simulink model "Simulink"  (R2023a)
settings: Solver=VariableStepAuto  StartTime=0.0  StopTime=1  RelTol=1e-3
libraries: dspmlti4 x10
settings Model: Creator=Hasan  LastModifiedBy=Hasan
settings DataIOCC: ReturnWorkspaceOutputs=off
settings DebuggingCC: ParameterPrecisionLossMsg=none

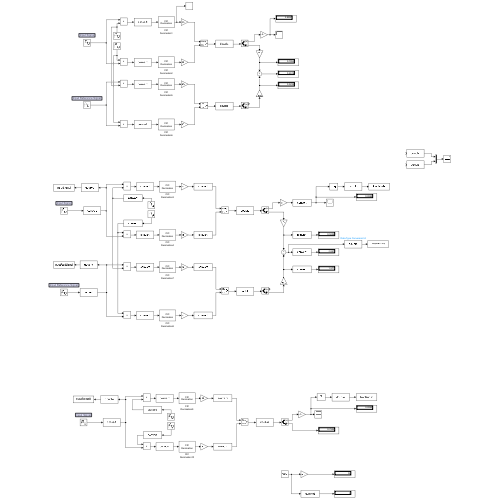
[thumbnail: Simulink's stored preview of the top-level diagram]
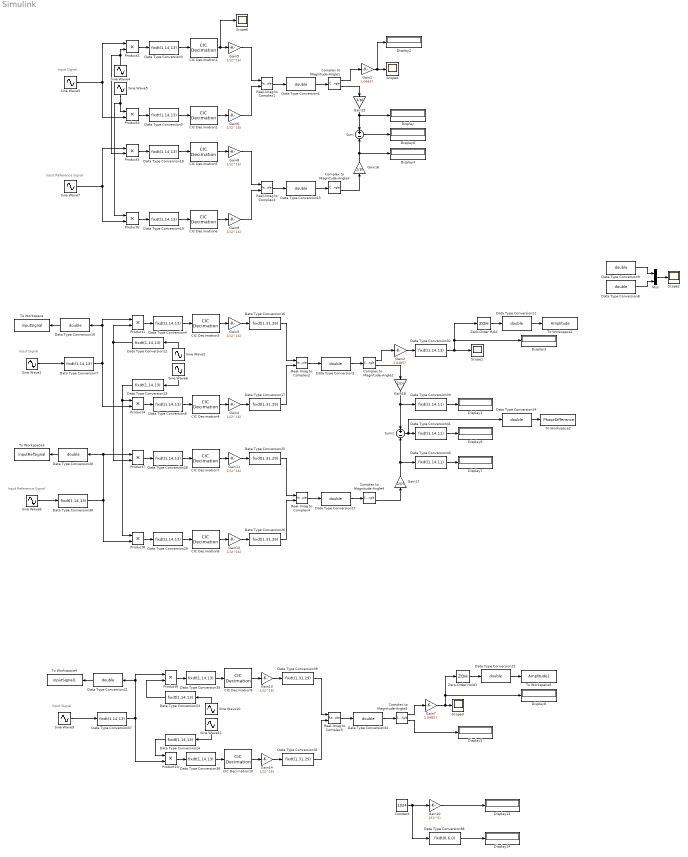
== system Simulink ==
  note: Input Signal
  note: Input Signal
  note: Input Reference Signal
  note: Input Reference Signal
  note: Input Signal
  CIC Decimation{1..2,4..6,8,10} (7 alike) : dspmlti4/CIC Decimation  filtFrom=Dialog parameters  filtobj=CICDECIM  ftype=Decimator  R=50  M=1  N=3  filterInternals=Full precision  BPS=[16 16 16 16]  FLPS=0  outputWordLength=50  outputFracLength=0  launchFVT=off  framing=Maintain input frame rate  RateOptions=Allow multirate processing
      settings: LibrarySourceBlock=|
      | dsphdlsupportfiltering/CIC
      | Decimation
  CIC Decimation3 : dspmlti4/CIC Decimation  filtFrom=Dialog parameters  filtobj=CICDECIM  ftype=Decimator  R=50  M=1  N=3  filterInternals=Full precision  BPS=[16 16 16 16]  FLPS=0  outputWordLength=14  outputFracLength=0  launchFVT=off  framing=Maintain input frame rate  RateOptions=Allow multirate processing
      settings: LibrarySourceBlock=|
      | dsphdlsupportfiltering/CIC
      | Decimation
  CIC Decimation7 : dspmlti4/CIC Decimation  filtFrom=Dialog parameters  filtobj=CICDECIM  ftype=Decimator  R=50  M=1  N=3  filterInternals=Full precision  BPS=[16 16 16 16]  FLPS=0  outputWordLength=14  outputFracLength=0  launchFVT=off  framing=Maintain input frame rate  RateOptions=Allow multirate processing
      settings: LibrarySourceBlock=|
      | dsphdlsupportfiltering/CIC
      | Decimation
  CIC Decimation9 : dspmlti4/CIC Decimation  filtFrom=Dialog parameters  filtobj=CICDECIM  ftype=Decimator  R=50  M=1  N=3  filterInternals=Full precision  BPS=[16 16 16 16]  FLPS=0  outputWordLength=14  outputFracLength=0  launchFVT=off  framing=Maintain input frame rate  RateOptions=Allow multirate processing
      settings: LibrarySourceBlock=|
      | dsphdlsupportfiltering/CIC
      | Decimation
  Complex to Magnitude-Angle{1..5} (5 alike) : ComplexToMagnitudeAngle
  Constant : Constant  Value=1024
  Data Type Conversion{1..2,8..11,14..15,20..22,27,34} (13 alike) : DataTypeConversion  OutDataTypeStr=double  SaturateOnIntegerOverflow=off  RndMeth=Floor
  Data Type Conversion{3..7,12..13,18..19,23..24,28..30,32,35..37} (18 alike) : DataTypeConversion  OutDataTypeStr=fixdt(1,14,13)  SaturateOnIntegerOverflow=off  RndMeth=Floor
  Data Type Conversion{16..17,25..26,31,39} (6 alike) : DataTypeConversion  OutDataTypeStr=fixdt(1,31,29)  SaturateOnIntegerOverflow=off  RndMeth=Floor
  Data Type Conversion33 : DataTypeConversion  OutDataTypeStr=fixdt(1,14,11)  SaturateOnIntegerOverflow=off  RndMeth=Floor
  Data Type Conversion38 : DataTypeConversion  OutDataTypeStr=fixdt(0,6,0)  SaturateOnIntegerOverflow=off  RndMeth=Floor
  Data Type Conversion40 : DataTypeConversion  OutDataTypeStr=fixdt(1,14,11)  SaturateOnIntegerOverflow=off  RndMeth=Floor
  Data Type Conversion41 : DataTypeConversion  OutDataTypeStr=fixdt(1,14,11)  SaturateOnIntegerOverflow=off  RndMeth=Floor
  Display{,1..9,13..14} (12 alike) : Display
  Gain1 : Gain  Gain=1.04857
  Gain10 : Gain  Gain=1/(2^5)  ParamDataTypeStr=double  OutDataTypeStr=double
  Gain{3..6,8..9,11..14} (10 alike) : Gain  Gain=1/(2^16)
  Gain15 : Gain  Gain=1/pi
  Gain16 : Gain  Gain=1/pi
  Gain17 : Gain  Gain=1/pi  ParamDataTypeStr=fixdt(1,14,12)  OutDataTypeStr=fixdt(1,29,25)
  Gain18 : Gain  Gain=1/pi  ParamDataTypeStr=fixdt(1,14,12)  OutDataTypeStr=fixdt(1,29,25)
  Gain2 : Gain  Gain=1.04857  ParamDataTypeStr=fixdt(1,14,12)  OutDataTypeStr=fixdt(1,29,25)
  Gain7 : Gain  Gain=1.04857  ParamDataTypeStr=fixdt(1,14,12)  OutDataTypeStr=fixdt(1,45,41)
  Mux : Mux  Inputs=2
  Product{1..10} (10 alike) : Product
  Real-Imag to Complex{1..5} (5 alike) : RealImagToComplex
  Scope{1..4,6} (5 alike) : Scope
  Sine Wave1 : Sin  Amplitude=.9  Frequency=2*pi*60e6  Phase=pi/6  SampleTime=1/150e6
  Sine Wave10 : Sin  Amplitude=0.9999  Frequency=2*pi*60e6  SampleTime=1/150e6
  Sine Wave11 : Sin  Amplitude=0.9999  Frequency=2*pi*60e6  Phase=pi/2  SampleTime=1/150e6
  Sine Wave2 : Sin  Amplitude=0.9999  Frequency=2*pi*60e6  SampleTime=1/150e6
  Sine Wave3 : Sin  Amplitude=0.9  Frequency=2*pi*60e6  Phase=pi/4  SampleTime=1/150e6
  Sine Wave4 : Sin  Amplitude=.9999  Frequency=2*pi*60e6  SampleTime=1/150e6
  Sine Wave5 : Sin  Amplitude=0.99999  Frequency=2*pi*60e6  Phase=pi/2  SampleTime=1/150e6
  Sine Wave6 : Sin  Amplitude=0.9999  Frequency=2*pi*60e6  Phase=pi/2  SampleTime=1/150e6
  Sine Wave7 : Sin  Amplitude=0.9  Frequency=2*pi*60e6  Phase=pi/6  SampleTime=1/150e6
  Sine Wave8 : Sin  Amplitude=0.9  Frequency=2*pi*60e6  Phase=pi/2  SampleTime=1/150e6
  Sine Wave9 : Sin  Amplitude=0.9  Frequency=2*pi*60e6  Phase=pi/4  SampleTime=1/150e6
  Sum : Sum  Inputs=+|-
  Sum1 : Sum  Inputs=+|-
  To Workspace : ToWorkspace  VariableName=inputSignal  SaveFormat=Timeseries  SampleTime=-1
  To Workspace1 : ToWorkspace  VariableName=Amplitude  SaveFormat=Timeseries  SampleTime=-1
  To Workspace2 : ToWorkspace  VariableName=PhaseDifference  SaveFormat=Timeseries  SampleTime=-1
  To Workspace3 : ToWorkspace  VariableName=inputRefSignal  SaveFormat=Timeseries  SampleTime=-1
  To Workspace4 : ToWorkspace  VariableName=inputSignal1  SaveFormat=Timeseries  SampleTime=-1
  To Workspace5 : ToWorkspace  VariableName=Amplitude1  SaveFormat=Timeseries  SampleTime=-1
  Zero-Order Hold : ZeroOrderHold  SampleTime=1/150e6
  Zero-Order Hold1 : ZeroOrderHold  SampleTime=1/150e6
  wires:
  Real-Imag to Complex1/1 -> Data Type Conversion1/1
  CIC Decimation1/1 -> Scope6/1, Gain5/1
  Sine Wave3/1 -> Product2/1, Product3/2
  Sine Wave4/1 -> Product5/2, Product2/2
  Product3/1 -> Data Type Conversion5/1
  Data Type Conversion3/1 -> CIC Decimation1/1
  Data Type Conversion5/1 -> CIC Decimation2/1
  CIC Decimation2/1 -> Gain6/1
  Data Type Conversion1/1 -> Complex to Magnitude-Angle1/1
  Complex to Magnitude-Angle1/1 -> Gain1/1
  Complex to Magnitude-Angle2/1 -> Gain2/1
  Data Type Conversion2/1 -> Complex to Magnitude-Angle2/1
  Data Type Conversion6/1 -> CIC Decimation4/1
  Data Type Conversion4/1 -> CIC Decimation3/1
  Product4/1 -> Data Type Conversion6/1
  Sine Wave6/1 -> Data Type Conversion13/1
  Real-Imag to Complex2/1 -> Data Type Conversion2/1
  Data Type Conversion7/1 -> Data Type Conversion10/1, Product1/1, Product4/2
  Data Type Conversion10/1 -> To Workspace/1
  Data Type Conversion11/1 -> To Workspace1/1
  Gain2/1 -> Data Type Conversion32/1
  Gain4/1 -> Data Type Conversion17/1
  Gain3/1 -> Data Type Conversion16/1
  Gain5/1 -> Real-Imag to Complex1/1
  Gain6/1 -> Real-Imag to Complex1/2
  Sine Wave2/1 -> Data Type Conversion12/1
  Data Type Conversion12/1 -> Product7/2, Product1/2
  Data Type Conversion13/1 -> Product8/1, Product4/1
  Data Type Conversion16/1 -> Real-Imag to Complex2/1
  Data Type Conversion17/1 -> Real-Imag to Complex2/2
  Product2/1 -> Data Type Conversion3/1
  Gain1/1 -> Display2/1, Scope4/1
  Zero-Order Hold/1 -> Data Type Conversion11/1
  CIC Decimation3/1 -> Gain3/1
  Product1/1 -> Data Type Conversion4/1
  CIC Decimation4/1 -> Gain4/1
  Complex to Magnitude-Angle1/2 -> Gain15/1
  Mux/1 -> Scope2/1
  Data Type Conversion8/1 -> Mux/2
  Data Type Conversion9/1 -> Mux/1
  Complex to Magnitude-Angle2/2 -> Gain18/1
  Data Type Conversion14/1 -> To Workspace2/1
  Sine Wave1/1 -> Data Type Conversion7/1
  Complex to Magnitude-Angle3/2 -> Gain16/1
  Product5/1 -> Data Type Conversion18/1
  Gain9/1 -> Real-Imag to Complex3/2
  Gain8/1 -> Real-Imag to Complex3/1
  Data Type Conversion15/1 -> Complex to Magnitude-Angle3/1
  CIC Decimation6/1 -> Gain9/1
  Data Type Conversion19/1 -> CIC Decimation6/1
  Data Type Conversion18/1 -> CIC Decimation5/1
  Product6/1 -> Data Type Conversion19/1
  Sine Wave7/1 -> Product6/2, Product5/1
  CIC Decimation5/1 -> Gain8/1
  Real-Imag to Complex3/1 -> Data Type Conversion15/1
  Sine Wave5/1 -> Product6/1, Product3/1
  Sum/1 -> Display6/1
  Sine Wave8/1 -> Data Type Conversion30/1
  Complex to Magnitude-Angle4/2 -> Gain17/1
  CIC Decimation8/1 -> Gain12/1
  Product7/1 -> Data Type Conversion28/1
  CIC Decimation7/1 -> Gain11/1
  Data Type Conversion26/1 -> Real-Imag to Complex4/2
  Data Type Conversion25/1 -> Real-Imag to Complex4/1
  Gain11/1 -> Data Type Conversion25/1
  Gain12/1 -> Data Type Conversion26/1
  Data Type Conversion20/1 -> To Workspace3/1
  Data Type Conversion30/1 -> Product7/1, Data Type Conversion20/1, Product8/2
  Real-Imag to Complex4/1 -> Data Type Conversion27/1
  Product8/1 -> Data Type Conversion29/1
  Data Type Conversion28/1 -> CIC Decimation7/1
  Data Type Conversion29/1 -> CIC Decimation8/1
  Data Type Conversion27/1 -> Complex to Magnitude-Angle4/1
  Data Type Conversion36/1 -> CIC Decimation10/1
  Data Type Conversion37/1 -> Data Type Conversion21/1, Product9/1, Product10/2
  Product10/1 -> Data Type Conversion36/1
  Sine Wave10/1 -> Data Type Conversion23/1
  Product9/1 -> Data Type Conversion35/1
  Data Type Conversion22/1 -> To Workspace5/1
  Zero-Order Hold1/1 -> Data Type Conversion22/1
  Sine Wave11/1 -> Data Type Conversion24/1
  Data Type Conversion23/1 -> Product9/2
  Data Type Conversion24/1 -> Product10/1
  Sine Wave9/1 -> Data Type Conversion37/1
  Real-Imag to Complex5/1 -> Data Type Conversion34/1
  Data Type Conversion35/1 -> CIC Decimation9/1
  Complex to Magnitude-Angle5/1 -> Gain7/1
  Data Type Conversion34/1 -> Complex to Magnitude-Angle5/1
  Data Type Conversion21/1 -> To Workspace4/1
  Complex to Magnitude-Angle5/2 -> Display5/1
  Gain7/1 -> Zero-Order Hold1/1, Display8/1, Scope3/1
  Constant/1 -> Data Type Conversion38/1, Gain10/1
  Gain10/1 -> Display13/1
  Data Type Conversion38/1 -> Display14/1
  CIC Decimation9/1 -> Gain13/1
  Gain13/1 -> Data Type Conversion39/1
  Data Type Conversion39/1 -> Real-Imag to Complex5/1
  Gain14/1 -> Data Type Conversion31/1
  CIC Decimation10/1 -> Gain14/1
  Data Type Conversion31/1 -> Real-Imag to Complex5/2
  Data Type Conversion32/1 -> Zero-Order Hold/1, Display3/1, Scope1/1
  Data Type Conversion33/1 -> Display1/1
  Data Type Conversion40/1 -> Display7/1
  Sum1/1 -> Data Type Conversion41/1, Data Type Conversion14/1
  Data Type Conversion41/1 -> Display9/1
  Gain15/1 -> Sum/1, Display/1
  Gain16/1 -> Sum/2, Display4/1
  Gain17/1 -> Data Type Conversion40/1, Sum1/2
  Gain18/1 -> Sum1/1, Data Type Conversion33/1
